simulink model "BLDC_HallSensor"  (R2023b)
settings: Solver=FixedStepAuto  StartTime=0.0  StopTime=10  FixedStep=1e-5  RelTol=1e-5
libraries: simulink x7, spsCurrentMeasurementLib x4, slpidlib x1, spsDCVoltageSourceLib x1, spsPermanentMagnetSynchronousMachineLib x1, spsUniversalBridgeLib x1, spsVoltageMeasurementLib x1, sps_lib x1
settings Model: Creator=84339  LastModifiedBy=84339
settings OptimizationCC: DefaultParameterBehavior=Inlined  EnhancedBackFolding=on  PassReuseOutputArgsAs=Individual arguments  ZeroExternalMemoryAtStartup=off  ZeroInternalMemoryAtStartup=off  OptimizeBlockOrder=speed  DifferentSizesBufferReuse=on  OptimizationCustomize=off  EfficientTunableParamExpr=on
settings DebuggingCC: ParameterTunabilityLossMsg=error
settings SFSimCC: MATLABDynamicMemAlloc=off
settings RTWCC: Description=Embedded Coder  SystemTargetFile=ert.tlc  GenCodeOnly=on  TemplateMakefile=ert_default_tmf
settings CodeAppCC: ForceParamTrailComments=on  IgnoreCustomStorageClasses=off  OperatorAnnotations=on  SimulinkDataObjDesc=on  SFDataObjDesc=on  InsertBlockDesc=on
settings ERTTargetCC: TargetLangStandard=C99 (ISO)  GenerateSampleERTMain=on  SupportContinuousTime=on  InlinedParameterPlacement=NonHierarchical  ERTCustomFileTemplate=example_file_process.tlc

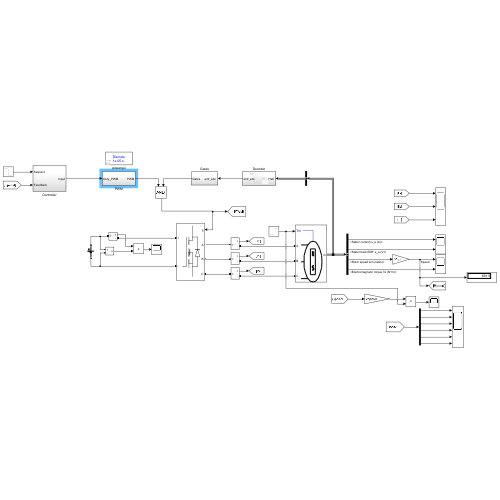
[thumbnail: Simulink's stored preview of the top-level diagram]
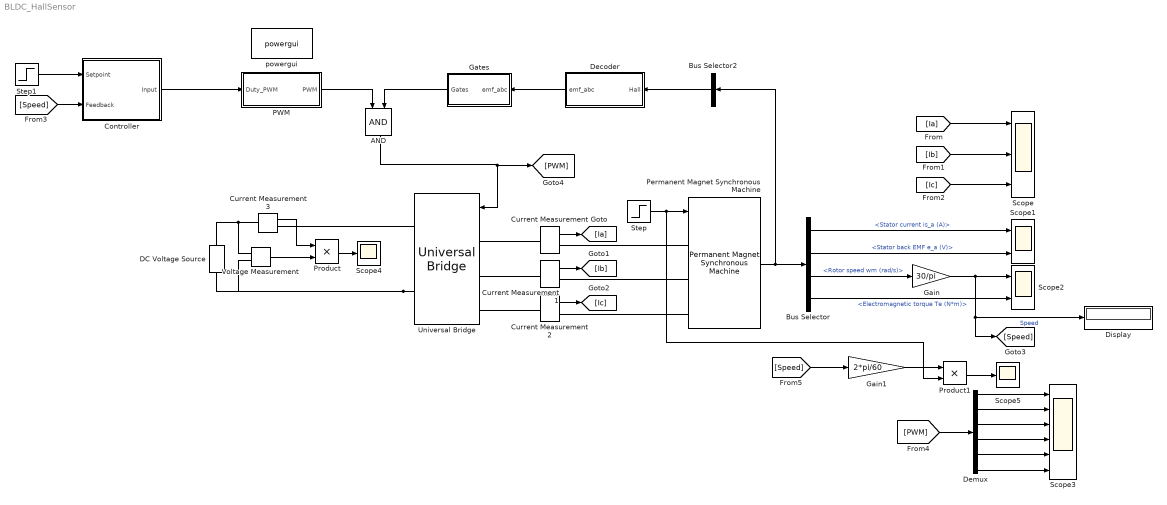
== system BLDC_HallSensor ==
  AND : Logic  AllPortsSameDT=off  OutDataTypeStr=boolean
  Bus Selector : BusSelector  OutputSignals=Stator current is_a (A),Stator back EMF e_a (V),Rotor speed wm (rad/s),Electromagnetic torque Te (N*m)
  Bus Selector2 : BusSelector  OutputSignals=Hall effect signal h_a,Hall effect signal h_b,Hall effect signal h_c  OutputAsBus=on
  Controller : Subsystem
  Current Measurement{,1..3} (4 alike) : spsCurrentMeasurementLib/Current Measurement  PhasorSimulation=off  OutputType=Complex  PSBequivalent=0
  DC Voltage Source : spsDCVoltageSourceLib/DC Voltage Source  Amplitude=100  Measurements=None
  Decoder : Subsystem
  Demux : Demux  Outputs=6
  Display : Display
  Gain : Gain  Gain=30/pi
  Gain1 : Gain  Gain=2*pi/60
  Gates : Subsystem
  PWM : Subsystem
  Permanent Magnet Synchronous Machine : spsPermanentMagnetSynchronousMachineLib/Permanent Magnet Synchronous Machine  NbPhases=3  FluxDistribution=Trapezoidal  RotorType=Round  MechanicalLoad=Torque Tm  PresetModel=No  ShowDetailedParameters=on  MeasurementBus=off  Resistance=0.0485  Inductance=8.5e-3  dqInductances=[8.5e-3,8.5e-3]  La=0.000395  MachineConstant=Flux linkage established by magnets (V.s)  Flux=0.1194  VoltageCst=100.0283  TorqueCst=0.9552  Flat=120  Mechanical=[0.0027 0.0004924 4 0]  PolePairs=4  InitialConditions=[0,0, 0,0]  InitialConditions5ph=[0 0 0 0 0 0]  RefAngle=90 degrees behind phase A axis (modified Park)  IterativeDiscreteModel=Trapezoidal non iterative  TsBlock=-1  TsPowergui=0
  Product : Product
  Product1 : Product
  Scope : Scope  NumInputPorts=3
  Scope1 : Scope  NumInputPorts=2
  Scope2 : Scope  NumInputPorts=2
  Scope3 : Scope  NumInputPorts=6
  Scope4 : Scope
  Scope5 : Scope
  Step : Step  Time=0  Before=10  After=10  SampleTime=0
  Step1 : Step  Time=3  Before=500  After=-500  SampleTime=0
  Universal Bridge : spsUniversalBridgeLib/Universal Bridge  Arms=3  SnubberResistance=5000  SnubberCapacitance=1e-6  Device=MOSFET / Diodes  Ron=1e-3  Lon=0  ForwardVoltages="[  0  0  ]"  ForwardVoltage=0  GTOparameters=[ 10e-6 , 20e-6 ]  IGBTparameters=[ 1e-6 , 2e-6 ]  Measurements=None  Measurements_2=None  converterType=Rectifier
  Voltage Measurement : spsVoltageMeasurementLib/Voltage Measurement  PhasorSimulation=off  OutputType=Complex  PSBequivalent=0
  powergui : sps_lib/powergui  Priority=1  SimulationMode=Discrete  SampleTime=1e-5  frequency=60  Iterations=50  frequencyindice=0  Pbase=100e6  ErrMax=1e-4  UnitsV=kV  UnitsW=MW  buscounter=0  FunctionMessages=off  echomessages=off  EnableUseOfTLC=off  CurrentSourceSwitches=off  DisableSnubberDevices=off  DisableRonSwitches=off  DisableVfSwitches=off  DisplayEquations=off  AutomaticDiscreteSolvers=off  SolverType=Tustin/Backward Euler (TBE)  Interpol=off  ExternalGateDelay=off  methode=off  Ts=100  x0status=blocks  SPID=on  SwTol=0  HookPort=off  NonlinearTolerance=1e-4  nMaxIteration=100  ContinueOnMaxIteration=off  RestoreLinks=warning  ResistiveCurrentMeasurement=off  Frange=[0:2:500]  Ylog=off  Xlog=on  ShowGrid=off  save=off  variable=ZData  structure=0  ZoomFFT=off  StartTime=0.0  cycles=1  DisplayStyle=1  fundamental=60  FreqAxis=off  MaxFrequency=1000  frequencyindicesteady=1  RmsSteady=1  display=off
  wires:
  Step/1 -> Product1/2, Permanent Magnet Synchronous Machine/1
  Current Measurement/1 -> [Ia]
  Current Measurement1/1 -> [Ib]
  Current Measurement2/1 -> [Ic]
  Permanent Magnet Synchronous Machine/1 -> Bus Selector2/1, Bus Selector/1
  Bus Selector2/1 -> Decoder/1("Hall ")
  [Ia] -> Scope/1
  [Ib] -> Scope/2
  [Ic] -> Scope/3
  Bus Selector/1 -> Scope1/1  "<Stator current is_a (A)>"
  Bus Selector/2 -> Scope1/2  "<Stator back EMF e_a (V)>"
  Bus Selector/3 -> Gain/1  "<Rotor speed wm (rad/s)>"
  Bus Selector/4 -> Scope2/2  "<Electromagnetic torque Te (N*m)>"
  Decoder/1(emf_abc) -> Gates/1("emf_abc ")
  Gates/1(Gates) -> AND/2
  PWM/1(PWM) -> AND/1
  Controller/1(Input) -> PWM/1(Duty_PWM)
  Gain/1 -> [Speed], Display/1, Scope2/1  "Speed"
  Step1/1 -> Controller/1(Setpoint)
  [Speed] -> Controller/2(Feedback)
  AND/1 -> Universal Bridge/1, [PWM]
  [PWM] -> Demux/1
  Demux/1 -> Scope3/1
  Demux/2 -> Scope3/2
  Demux/3 -> Scope3/3
  Demux/4 -> Scope3/4
  Demux/5 -> Scope3/5
  Demux/6 -> Scope3/6
  Current Measurement3/1 -> Product/1
  Voltage Measurement/1 -> Product/2
  Product/1 -> Scope4/1
  [Speed] -> Gain1/1
  Gain1/1 -> Product1/1
  Product1/1 -> Scope5/1
  connections:
  Universal Bridge/LConn1 -- Current Measurement/LConn1
  Current Measurement1/LConn1 -- Universal Bridge/LConn2
  Universal Bridge/LConn3 -- Current Measurement2/LConn1
  Current Measurement/RConn1 -- Permanent Magnet Synchronous Machine/LConn1
  Current Measurement1/RConn1 -- Permanent Magnet Synchronous Machine/LConn2
  Current Measurement2/RConn1 -- Permanent Magnet Synchronous Machine/LConn3
  Universal Bridge/RConn2 -- DC Voltage Source/LConn1 -- Voltage Measurement/LConn2
  Current Measurement3/LConn1 -- DC Voltage Source/RConn1 -- Voltage Measurement/LConn1
  Current Measurement3/RConn1 -- Universal Bridge/RConn1

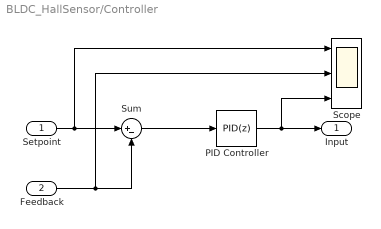
== system BLDC_HallSensor/Controller ==
  Setpoint : Inport
  Feedback : Inport  Port=2
  PID Controller : slpidlib/PID Controller  Controller=PID  Form=Parallel  TimeDomain=Discrete-time  UseExternalTs=off  SampleTime=1e-5  IntegratorMethod=Forward Euler  FilterMethod=Forward Euler  ControllerParametersSource=internal  P=0.4  I=0.3  UseKiTs=off  D=0.03  N=100  UseFilter=off  TunerSelectOption=Frequency Response Based  InitialConditionSource=internal  InitialConditionForIntegrator=0  InitialConditionForFilter=0  DifferentiatorICPrevScaledInput=0  ExternalReset=none  TrackingMode=off  Kt=1  LimitOutput=on  SatLimitsSource=internal  UpperSaturationLimit=100  LowerSaturationLimit=-100  LinearizeAsGain=on  AntiWindupMode=none  Kb=1  LimitIntegrator=off  UpperIntegratorSaturationLimit=inf  LowerIntegratorSaturationLimit=-inf  POutMin=[]  POutMax=[]  IOutMin=[]  IOutMax=[]  DOutMin=[]  DOutMax=[]  NOutMin=[]  NOutMax=[]  SumOutMin=[]  SumOutMax=[]  SaturationOutMin=[]  SaturationOutMax=[]  PParamMin=[]  PParamMax=[]  IParamMin=[]  IParamMax=[]  DParamMin=[]  DParamMax=[]  NParamMin=[]  NParamMax=[]  KbParamMin=[]  KbParamMax=[]  KtParamMin=[]  KtParamMax=[]  KbOutMin=[]  KbOutMax=[]  KtOutMin=[]  KtOutMax=[]  IntegratorOutMin=[]  IntegratorOutMax=[]  FilterOutMin=[]  FilterOutMax=[]  SumI1OutMin=[]  SumI1OutMax=[]  SumI2OutMin=[]  SumI2OutMax=[]  SumI3OutMin=[]  SumI3OutMax=[]  SumI4OutMin=[]  SumI4OutMax=[]  SumDOutMin=[]  SumDOutMax=[]  DifferentiatorOutMin=[]  DifferentiatorOutMax=[]  FilterDiffOutCoefMin=[]  FilterDiffOutCoefMax=[]  ReciprocalOutMin=[]  ReciprocalOutMax=[]  SumDenOutMin=[]  SumDenOutMax=[]  SumNumOutMin=[]  SumNumOutMax=[]  DivideOutMin=[]  DivideOutMax=[]  UdiffTsProdOutMin=[]  UdiffTsProdOutMax=[]  NTsProdOutMin=[]  NTsProdOutMax=[]  UintegralTsProdOutMin=[]  UintegralTsProdOutMax=[]  UngainTsProdOutMin=[]  UngainTsProdOutMax=[]  ClampingZeroOutDataTypeStr=Inherit: Inherit via back propagation  ClampingZeroOutMin=[]  ClampingZeroOutMax=[]  FilterDenConstantOutDataTypeStr=Inherit: Inherit via back propagation  FilterDenConstantOutMin=[]  FilterDenConstantOutMax=[]  PCopyOutDataTypeStr=Inherit: Inherit via back propagation  PCopyOutMin=[]  PCopyOutMax=[]  NCopyOutDataTypeStr=Inherit: Inherit via back propagation  NCopyOutMin=[]  NCopyOutMax=[]  IntegratorContinuousStateAttributes=''  IntegratorStateMustResolveToSignalObject=off  IntegratorRTWStateStorageClass=Auto  FilterContinuousStateAttributes=''  FilterStateMustResolveToSignalObject=off  FilterRTWStateStorageClass=Auto  ParallelPVariant=InternalParameters  IdealPVariant=Disabled  IVariant=InternalParameters  DVariant=InternalParameters  IntegratorVariant=Discrete  SatVariant=Enabled  AWVariant=Passthrough  PCopyVariant=Disabled  TRVariant=Disabled  FdbkBlocksVariant=Forward  IdealPFdbkVariant=Disabled  SatFdbkVariant=Disabled  DerivativeFilterVariant=Differentiator  NVariant=Passthrough  NCopyVariant=Disabled_SignalSpec  FilterICVariant=InternalICsDifferentiator  IntegratorICVariant=InternalICs  ExternalResetVariant=Disabled  TRSumVariant=Passthrough  SumFdbkVariant=Disabled  SumVariant=Sum_PID  TsampFilterVariant=InternalTs  TsampNgainVariant=Passthrough  TsampIntegralVariant=Disabled_SignalSpec  ExternalSaturationOutDataTypeStr=Inherit: Same as second input
  Scope : Scope  NumInputPorts=3
  Sum : Sum  Inputs=|+-
  Input : Outport
  wires:
  Sum/1 -> PID Controller/1
  Feedback/1 -> Scope/2, Sum/2
  Setpoint/1 -> Scope/1, Sum/1
  PID Controller/1 -> Scope/3, Input/1

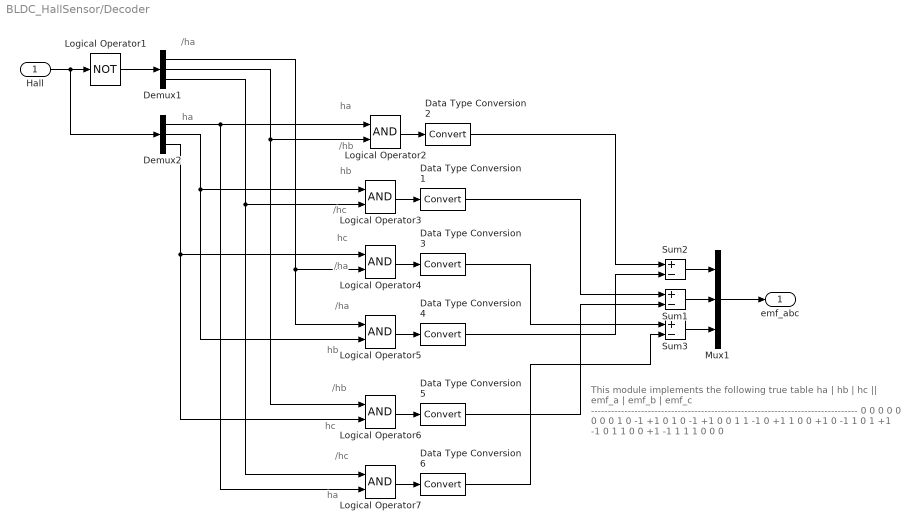
== system BLDC_HallSensor/Decoder ==
  note: This module implements the following true table
      |
      |    ha   |   hb   |   hc   ||   emf_a   |   emf_b   |   emf_c
      |     --------------------------------------------------------------------------------
      | 0          0         0          0               0               0
      | 0          0         1          0               -1              +1
      | 0          1         0          -1              +1                0
      | 0          1         1          -1               0               +1
      | 1          0         0         +1               0               -1
      | 1          0         1         +1              -1                0
      | 1          1         0          0              +1               -1
      | 1          1         1          0               0                0
  note: ha
  note: /ha
  note: /ha
  note: ha
  note: /ha
  note: /hc
  note: /hb
  note: /hb
  note: hb
  note: hb
  note: hc
  note: hc
  note: ha
  note: /hc
  "Hall " : Inport
  Data Type Conversion{1..6} (6 alike) : DataTypeConversion  SaturateOnIntegerOverflow=off  RndMeth=Floor
  Demux1 : Demux  Outputs=3
  Demux2 : Demux  Outputs=3
  Logical Operator1 : Logic  Operator=NOT  AllPortsSameDT=off  OutDataTypeStr=boolean
  Logical Operator{2..7} (6 alike) : Logic  AllPortsSameDT=off  OutDataTypeStr=boolean
  Mux1 : Mux  Inputs=3
  Sum1 : Sum  Inputs=+-  OutDataTypeStr=double
  Sum2 : Sum  Inputs=+-  OutDataTypeStr=double
  Sum3 : Sum  Inputs=+-  OutDataTypeStr=double
  emf_abc : Outport
  wires:
  Demux2/3 -> Logical Operator4/1, Logical Operator6/2
  Data Type Conversion1/1 -> Sum1/1
  Logical Operator3/1 -> Data Type Conversion1/1
  Data Type Conversion6/1 -> Sum3/2
  Data Type Conversion4/1 -> Sum2/2
  Logical Operator6/1 -> Data Type Conversion5/1
  Mux1/1 -> emf_abc/1
  Demux1/1 -> Logical Operator4/2, Logical Operator5/1
  Sum3/1 -> Mux1/3
  Demux2/1 -> Logical Operator2/1, Logical Operator7/2
  Data Type Conversion2/1 -> Sum2/1
  Data Type Conversion5/1 -> Sum1/2
  "Hall "/1 -> Logical Operator1/1, Demux2/1
  Logical Operator2/1 -> Data Type Conversion2/1
  Logical Operator7/1 -> Data Type Conversion6/1
  Data Type Conversion3/1 -> Sum3/1
  Demux2/2 -> Logical Operator3/1, Logical Operator5/2
  Logical Operator5/1 -> Data Type Conversion4/1
  Sum2/1 -> Mux1/1
  Logical Operator4/1 -> Data Type Conversion3/1
  Sum1/1 -> Mux1/2
  Logical Operator1/1 -> Demux1/1
  Demux1/2 -> Logical Operator2/2, Logical Operator6/1
  Demux1/3 -> Logical Operator3/2, Logical Operator7/1

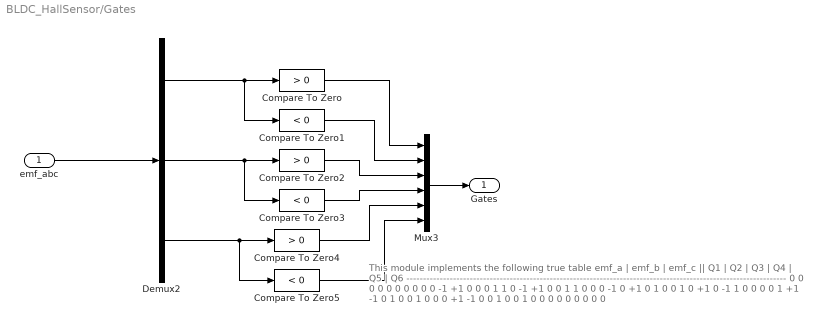
== system BLDC_HallSensor/Gates ==
  note: This module implements the following true table
      |
      |    emf_a   |   emf_b   |   emf_c   ||   Q1   |   Q2   |   Q3   |   Q4   |   Q5   |   Q6
      |     ------------------------------------------------------------------------------------------------------------------
      |       0              0                0            0          0          0           0        0        0
      |       0               -1              +1          0          0          0           1        1        0
      |     -1              +1                0          0          1          1           0        0        0
      |     -1               0               +1          0          1         0           0        1        0
      |    +1               0                -1          1          0          0           0        0        1
      |    +1              -1                0           1          0          0           1        0        0
      |      0              +1               -1           0          0          1           0        0        1
      |     0              0                0             0          0          0           0        0        0
  "emf_abc " : Inport
  Compare To Zero : simulink/Logic and Bit Operations/Compare To Zero  relop=>  OutDataTypeStr=boolean  ZeroCross=off
  Compare To Zero1 : simulink/Logic and Bit Operations/Compare To Zero  relop=<  OutDataTypeStr=boolean  ZeroCross=off
  Compare To Zero2 : simulink/Logic and Bit Operations/Compare To Zero  relop=>  OutDataTypeStr=boolean  ZeroCross=off
  Compare To Zero3 : simulink/Logic and Bit Operations/Compare To Zero  relop=<  OutDataTypeStr=boolean  ZeroCross=off
  Compare To Zero4 : simulink/Logic and Bit Operations/Compare To Zero  relop=>  OutDataTypeStr=boolean  ZeroCross=off
  Compare To Zero5 : simulink/Logic and Bit Operations/Compare To Zero  relop=<  OutDataTypeStr=boolean  ZeroCross=off
  Demux2 : Demux  Outputs=3
  Mux3 : Mux  Inputs=6
  Gates : Outport
  wires:
  "emf_abc "/1 -> Demux2/1
  Mux3/1 -> Gates/1
  Demux2/1 -> Compare To Zero/1, Compare To Zero1/1
  Demux2/2 -> Compare To Zero2/1, Compare To Zero3/1
  Demux2/3 -> Compare To Zero4/1, Compare To Zero5/1
  Compare To Zero/1 -> Mux3/1
  Compare To Zero1/1 -> Mux3/2
  Compare To Zero2/1 -> Mux3/3
  Compare To Zero3/1 -> Mux3/4
  Compare To Zero4/1 -> Mux3/5
  Compare To Zero5/1 -> Mux3/6

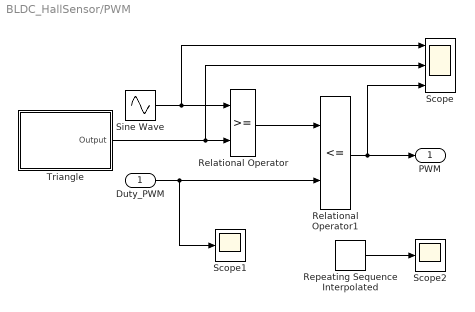
== system BLDC_HallSensor/PWM ==
  Duty_PWM : Inport
  Relational Operator : RelationalOperator  OutDataTypeStr=boolean  RndMeth=Simplest  InputSameDT=off
  Relational Operator1 : RelationalOperator  Operator=<=  OutDataTypeStr=boolean  RndMeth=Simplest  InputSameDT=off
  Repeating Sequence Interpolated : simulink/Sources/Repeating Sequence Interpolated  OutValues=[-1 1 -1]  TimeValues=[0 5e-4 1e-3]  LookUpMeth=Interpolation-Use End Values  tsamp=1e-5  OutMin=[]  OutMax=[]  OutDataTypeStr=single  OutputDataTypeScalingMode=single  OutDataType=fixdt(0,8)  OutScaling=2^-10
  Scope : Scope  NumInputPorts=3
  Scope1 : Scope
  Scope2 : Scope
  Sine Wave : Sin  Frequency=50*2*pi  SampleTime=0
  Triangle : Subsystem
  PWM : Outport
  wires:
  Sine Wave/1 -> Scope/1, Relational Operator/1
  Triangle/1(Output) -> Relational Operator/2, Scope/2
  Duty_PWM/1 -> Scope1/1, Relational Operator1/2
  Relational Operator/1 -> Relational Operator1/1
  Relational Operator1/1 -> Scope/3, PWM/1
  Repeating Sequence Interpolated/1 -> Scope2/1

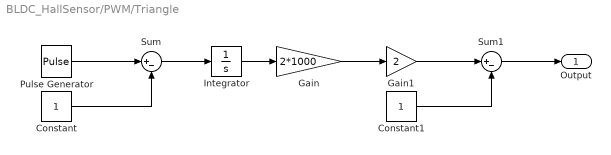
== system BLDC_HallSensor/PWM/Triangle ==
  Constant : Constant
  Constant1 : Constant
  Gain : Gain  Gain=2*1000
  Gain1 : Gain  Gain=2
  Integrator : Integrator
  Pulse Generator : DiscretePulseGenerator  PulseType=Time based  Amplitude=2  Period=1/1000  PulseWidth=50
  Sum : Sum  Inputs=|+-
  Sum1 : Sum  Inputs=|+-
  Output : Outport
  wires:
  Sum/1 -> Integrator/1
  Integrator/1 -> Gain/1
  Constant/1 -> Sum/2
  Pulse Generator/1 -> Sum/1
  Sum1/1 -> Output/1
  Gain/1 -> Gain1/1
  Gain1/1 -> Sum1/1
  Constant1/1 -> Sum1/2
